simulink model "Autonomous_4x4_ML_Control"  (R2026a)
settings: Solver=FixedStepAuto  StopTime=10  FixedStep=0.01  MaxStep=.01  AbsTol=1e-6
PreLoadFcn:
  | % Load initialization data
  | 
  | sldemo_absdata;
undefined symbols (not defined in the file): DiscIntNeverNeededParam, g, m, m_vehicle, mu, RoadFrictionFactor, Rr, slip, v0
libraries: statsLibrary x1
CloseFcn:
  | % Close the plots that are still open
  | h = findobj(0, 'Name', 'ABS Speeds');
  | if ~isempty(h),
  |   close(h);
  | end;
  | 
  | h = findobj(0, 'Name', 'ABS Slip');
  | if ~isempty(h),
  |   close(h);
  | end;
  | 
  | % Clear initial conditions data to avoid cluttering the workspace
  | 
  | clear g v0 Rr Kf m PBmax TB I slip mu ctrl h;
Description:
  | Modeling an Anti-Lock Braking System (ABS)
  | 
  | *Summary*
  | 
  | This example describes a simple model for an Anti-Lock Braking System
  | (ABS). The model simulates the dynamic behavior of a vehicle
  | under hard braking conditions. The model represents a single wheel, which
  | may be replicated a number of times to create a model for a multi-wheel
  | vehicle.
  | 
  | This model uses the signal logging feature in Simulink(R). You log signals to the
  | MATLAB(R) workspace where you can analyze and view them. You can view
  | the code in sldemo_absbrakeplots.m to see how this is done.
  | 
  | In this model, the wheel speed is calculated in a separate component
  | named sldemo_wheelspeed_absbrake.
  | This component is then referenced using a Model block.  Note that both the
  | top model and the referenced model use a variable step solver, so Simulink
  | will track zero-crossings in the referenced model.
settings Model: FPTRunName=Active  ModifiedByFormat=The MathWorks, Inc.  ExtModeTrigMode=oneshot  ExtModeArmWhenConnect=off  ExtModeAutoUpdateStatusClock=off  Creator=The MathWorks, Inc.  LastModifiedBy=The MathWorks, Inc.
settings DataIOCC: TimeSaveName=time  SignalLoggingName=sldemo_absbrake_output
settings OptimizationCC: UseDivisionForNetSlopeComputation=on  InlineInvariantSignals=on  StateBitsets=on  DataBitsets=on  EfficientFloat2IntCast=on  BufferReusableBoundary=off
settings DebuggingCC: SignalInfNanChecking=warning  SaveWithParameterizedLinksMsg=none  SigSpecEnsureSampleTimeMsg=none  IntegerOverflowMsg=error  UniqueDataStoreMsg=error  BusObjectLabelMismatch=none  AssertControl=DisableAll  SubsystemReferenceDiagnosticForUnitTest=warning  SFUndirectedBroadcastEventsDiag=error  IntegerSaturationMsg=none
settings HardwareCC: ProdHWDeviceType=32-bit Generic  TargetBitPerPointer=64.0  TargetBitPerSizeT=64.0  TargetBitPerPtrDiffT=64.0  TargetLongLongMode=on  TargetIntDivRoundTo=Zero  TargetEndianess=LittleEndian  TargetWordSize=64.0  TargetHWDeviceType=MATLAB Host
settings SFSimCC: CompileTimeRecursionLimit=0.0  EnableRuntimeRecursion=off
settings RTWCC: SystemTargetFile=ert.tlc  Description=Embedded Coder
settings CodeAppCC: IgnoreTestpoints=on  MATLABFcnDesc=on
settings ERTTargetCC: EnableSignedLeftShifts=off  EnableSignedRightShifts=off  DynamicArrayContainerType=coder::array  UtilityFuncGeneration=Shared location  GenerateSampleERTMain=on  SupportAbsoluteTime=off  ParenthesesLevel=Standards  CastingMode=Standards  GenerateSharedConstants=off
settings SimscapeCC: SimscapeLogType=none  SimscapeNominalValues="[{\"value\":\"1\",\"unit\":\"A\"},{\"value\":\"1\",\"unit\":\"bar\"},{\"value\":\"1\",\"unit\":\"cm^2\"},{\"value\":\"1\",\"unit\":\"cm^3/s\"},{\"value\":\"1\",\"unit\":\"kJ/kg\"},{\"value\":\"1\",\"unit\":\"kW\"},{\"value\":\"1\",\"unit\":\"l\"},{\"value\":\"1\",\"unit\":\"N\"},{\"value\":\"1\",\"unit\":\"N*m\"},{\"value\":\"1\",\"unit\":\"V\"}]"  SimscapeLogDataHistory=5000.0

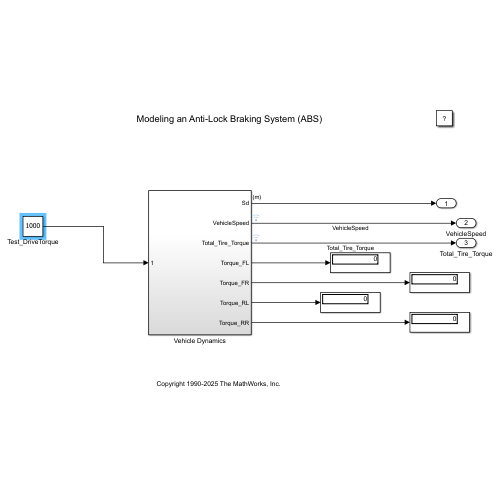
[thumbnail: Simulink's stored preview of the top-level diagram]
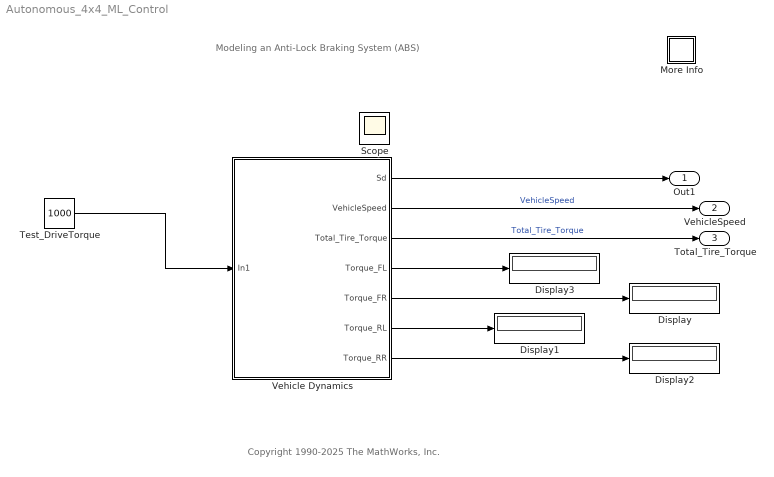
== system Autonomous_4x4_ML_Control ==
  note: Modeling an Anti-Lock Braking System (ABS)
  note: Copyright 1990-2025 The MathWorks, Inc.
  Display{,1..3} (4 alike) : Display
  More Info : Subsystem
      settings: OpenFcn=showExample('simulink_automotive/ModelingAnAntiLockBrakingSystemExample')
      mask Display: disp('?')
  Test_DriveTorque : Constant  Value=1000
  Vehicle Dynamics : Subsystem
  Out1 : Outport
  VehicleSpeed : Outport  Port=2
  Total_Tire_Torque : Outport  Port=3
  Scope : Scope
      settings: ActiveDisplayYMinimum=-8.8  ActiveDisplayYMaximum=79.2
  wires:
  Vehicle Dynamics/1(Sd) -> Out1/1
  Vehicle Dynamics/2(VehicleSpeed) -> VehicleSpeed/1  "VehicleSpeed"
  Vehicle Dynamics/3(Total_Tire_Torque) -> Total_Tire_Torque/1  "Total_Tire_Torque"
  Test_DriveTorque/1 -> Vehicle Dynamics/1(In1)
  Vehicle Dynamics/5(Torque_FR) -> Display/1
  Vehicle Dynamics/4(Torque_FL) -> Display3/1
  Vehicle Dynamics/6(Torque_RL) -> Display1/1
  Vehicle Dynamics/7(Torque_RR) -> Display2/1

== system Autonomous_4x4_ML_Control/More Info ==

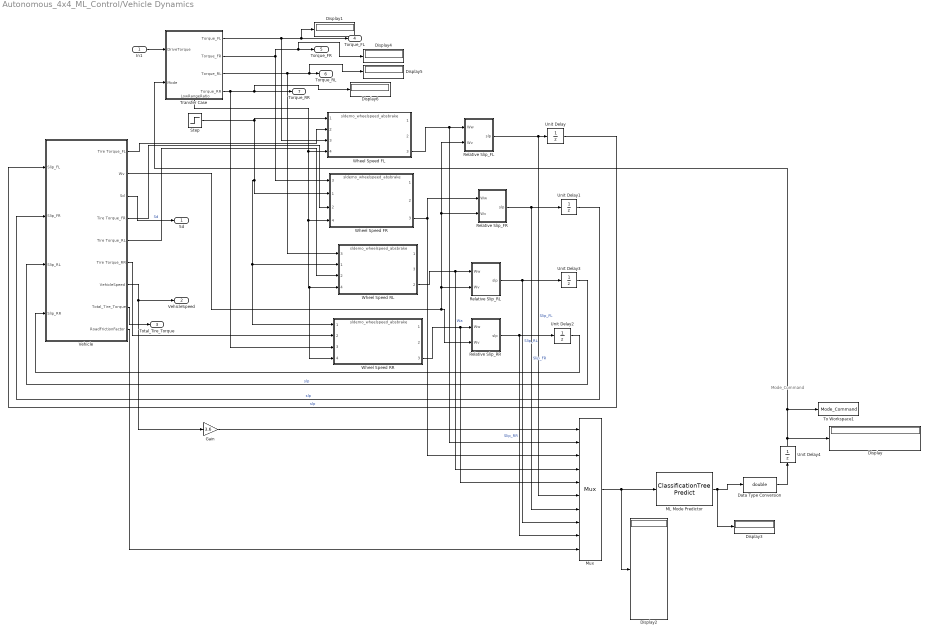
== system Autonomous_4x4_ML_Control/Vehicle Dynamics ==
  note: Mode_Command
  In1 : Inport
  Data Type Conversion : DataTypeConversion  OutDataTypeStr=double  SaturateOnIntegerOverflow=off  RndMeth=Floor
  Display{,1..6} (7 alike) : Display
  Gain : Gain  Gain=3.6
  ML Mode Predictor : statsLibrary/Classification/ClassificationTree Predict  TrainedLearner=MdlNum  ShowOutputScore=off  LabelDataTypeStr=Inherit: Inherit via back propagation  LabelOutMin=[]  LabelOutMax=[]  ScoreOutMin=[]  ScoreOutMax=[]  RawScoreOutMin=[]  RawScoreOutMax=[]  StoredEnumName=Mdl_enumLabels
  Mux : Mux  Inputs=10
  Relative Slip_FL : Subsystem
  Relative Slip_FR : Subsystem
  Relative Slip_RL : Subsystem
  Relative Slip_RR : Subsystem
  Step : Step  FinalValue=0  SampleTime=0
  To Workspace1 : ToWorkspace  VariableName=Mode_Command  SaveFormat=Timeseries  SampleTime=-1
  Transfer Case : Subsystem
      settings: PortSchema="{\"entries\":[{\"content\":{\"sides\":[{\"content\":{\"connectorIds\":[\"In1\",\"In2\"]},\"type\":\"ConnectorPlacement.EquallySpacedRectSide\",\"uuid\":\"0e4e5f2d-5f0e-4b2d-8d61-bd21c92eebc1\"},{\"content\":{\"connectorIds\":[\"Out1\",\"Out2\",\"Out3\",\"Out4\"],\"side\":\"RIGHT\"},\"type\":\"ConnectorPlacement.EquallySpacedRectSide\",\"uuid\":\"021f75cc-2385-4e1f-b164-196169dc630e\"},{\"content\":{\"side\":\"TOP\"},\"type\":\"ConnectorPlacement.EquallySpacedRectSide\",\"uuid\":\"94e51013-e54e-4a02-821d-d2a992c60f52\"},{\"content\":{\"connectorIds\":[\"Out5\"],\"side\":\"BOTTOM\"},\"type\":\"ConnectorPlacement.EquallySpacedRectSide\",\"uuid\":\"7324c2ae-c4f9-4421-b606-f82c567ae911\"}]},\"type\":\"ConnectorPlacement.EquallySpacedConnector\",\"uuid\":\"f212706d-3322-46ed-bdef-506210d0e9a5\"}],\"packageUris\":[\"http://schema.mathworks.com/mf0/Connector/R2020b\"],\"version\":\"1.0\"}"
  Unit Delay{,1..3} (4 alike) : UnitDelay  SampleTime=-1
  Unit Delay4 : UnitDelay  InitialCondition=1  SampleTime=-1
  "Vehicle  " : Subsystem
  Wheel Speed FL : ModelReference  ModelNameDialog=sldemo_wheelspeed_absbrake.slx  SimulationMode=Normal  ModelReferenceVersion=12.11
  Wheel Speed FR : ModelReference  ModelNameDialog=sldemo_wheelspeed_absbrake.slx  SimulationMode=Normal  ModelReferenceVersion=12.11
      settings: PortSchema="{\"entries\":[{\"content\":{\"sides\":[{\"content\":{\"connectorIds\":[\"In3\",\"In1\",\"In2\",\"In4\"]},\"type\":\"ConnectorPlacement.EquallySpacedRectSide\",\"uuid\":\"6283c4c6-a8cc-4cb2-bc3f-0488b786ccc3\"},{\"content\":{\"connectorIds\":[\"Out1\",\"Out2\",\"Out3\"],\"side\":\"RIGHT\"},\"type\":\"ConnectorPlacement.EquallySpacedRectSide\",\"uuid\":\"a506e2fe-25e7-45ab-91bb-1a7478d37f38\"},{\"content\":{\"side\":\"TOP\"},\"type\":\"ConnectorPlacement.EquallySpacedRectSide\",\"uuid\":\"8c371bb1-0729-467b-a425-cd217e166b59\"}]},\"type\":\"ConnectorPlacement.EquallySpacedConnector\",\"uuid\":\"2368ccbb-17fd-4c6b-9b61-3c68c899a72d\"}],\"packageUris\":[\"http://schema.mathworks.com/mf0/Connector/R2020b\"],\"version\":\"1.0\"}"
  Wheel Speed RL : ModelReference  ModelNameDialog=sldemo_wheelspeed_absbrake.slx  SimulationMode=Normal  ModelReferenceVersion=12.11
      settings: PortSchema="{\"entries\":[{\"content\":{\"sides\":[{\"content\":{\"connectorIds\":[\"In3\",\"In1\",\"In2\",\"In4\"]},\"type\":\"ConnectorPlacement.EquallySpacedRectSide\",\"uuid\":\"6283c4c6-a8cc-4cb2-bc3f-0488b786ccc3\"},{\"content\":{\"connectorIds\":[\"Out1\",\"Out3\",\"Out2\"],\"side\":\"RIGHT\"},\"type\":\"ConnectorPlacement.EquallySpacedRectSide\",\"uuid\":\"a506e2fe-25e7-45ab-91bb-1a7478d37f38\"},{\"content\":{\"side\":\"TOP\"},\"type\":\"ConnectorPlacement.EquallySpacedRectSide\",\"uuid\":\"8c371bb1-0729-467b-a425-cd217e166b59\"}]},\"type\":\"ConnectorPlacement.EquallySpacedConnector\",\"uuid\":\"2368ccbb-17fd-4c6b-9b61-3c68c899a72d\"}],\"packageUris\":[\"http://schema.mathworks.com/mf0/Connector/R2020b\"],\"version\":\"1.0\"}"
  Wheel Speed RR : ModelReference  ModelNameDialog=sldemo_wheelspeed_absbrake.slx  SimulationMode=Normal  ModelReferenceVersion=12.11
  Sd : Outport
  VehicleSpeed : Outport  Port=2
  Total_Tire_Torque : Outport  Port=3
  Torque_FL : Outport  Port=4
  Torque_FR : Outport  Port=5
  Torque_RL : Outport  Port=6
  Torque_RR : Outport  Port=7
  wires:
  "Vehicle  "/2(Wv) -> Relative Slip_RR/2(Wv), Relative Slip_RL/2(Wv), Relative Slip_FR/2(Wv), Relative Slip_FL/2(Wv)
  "Vehicle  "/1(Tire Torque_FL) -> Wheel Speed FL/2
  "Vehicle  "/3(Sd) -> Sd/1  "Sd"
  Relative Slip_FL/1(slp) -> Mux/6, Unit Delay/1  "Slip_FL"
  Unit Delay2/1 -> "Vehicle  "/4(Slip_RR)
  "Vehicle  "/4(Tire Torque_FR) -> Wheel Speed FR/2
  "Vehicle  "/5(Tire Torque_RL) -> Wheel Speed RL/2
  "Vehicle  "/6(Tire Torque_RR) -> Wheel Speed RR/2
  Relative Slip_FR/1(slp) -> Mux/7, Unit Delay1/1  "Slip_FR"
  Relative Slip_RL/1(slp) -> Mux/8, Unit Delay3/1  "Slip_RL"
  Relative Slip_RR/1(slp) -> Mux/9, Unit Delay2/1  "Slip_RR"
  Unit Delay/1 -> "Vehicle  "/1(Slip_FL)  "slp"
  Unit Delay1/1 -> "Vehicle  "/2(Slip_FR)  "slp"
  Unit Delay3/1 -> "Vehicle  "/3(Slip_RL)  "slp"
  Step/1 -> Wheel Speed RR/1, Wheel Speed RL/1, Wheel Speed FR/1, Wheel Speed FL/1
  "Vehicle  "/7(VehicleSpeed) -> VehicleSpeed/1, Gain/1
  "Vehicle  "/8(Total_Tire_Torque) -> Total_Tire_Torque/1
  In1/1 -> Transfer Case/1(DriveTorque)
  Transfer Case/1(Torque_FL) -> Display1/1, Torque_FL/1, Wheel Speed FL/3
  Transfer Case/2(Torque_FR) -> Display4/1, Torque_FR/1, Wheel Speed FR/3
  Transfer Case/3(Torque_RL) -> Wheel Speed RL/3, Display5/1, Torque_RL/1
  Transfer Case/4(Torque_RR) -> Wheel Speed RR/3, Display6/1, Torque_RR/1
  Transfer Case/5(LowRangeRatio) -> Wheel Speed RR/4, Wheel Speed RL/4, Wheel Speed FR/4, Wheel Speed FL/4
  Gain/1 -> Mux/1
  Wheel Speed FL/3 -> Mux/2, Relative Slip_FL/1(Ww)
  Wheel Speed FR/3 -> Mux/3, Relative Slip_FR/1(Ww)
  Wheel Speed RL/2 -> Mux/4, Relative Slip_RL/1(Ww)  "Wa"
  Wheel Speed RR/3 -> Mux/5, Relative Slip_RR/1(Ww)
  Mux/1 -> Display2/1, ML Mode Predictor/1
  "Vehicle  "/9(RoadFrictionFactor) -> Mux/10
  ML Mode Predictor/1 -> Display3/1, Data Type Conversion/1
  Data Type Conversion/1 -> Unit Delay4/1
  Unit Delay4/1 -> To Workspace1/1, Transfer Case/2(Mode), Display/1

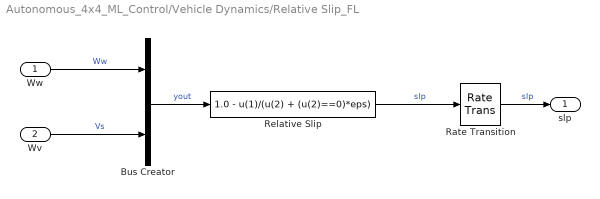
== system Autonomous_4x4_ML_Control/Vehicle Dynamics/Relative Slip_FL ==
  Ww : Inport
  Wv : Inport  Port=2
  Bus Creator : BusCreator  Inputs=2
  Rate Transition : RateTransition  OutPortSampleTimeOpt=Inherit
  Relative Slip : Fcn  Expr=1.0 - u(1)/(u(2) + (u(2)==0)*eps)
  slp : Outport
  wires:
  Bus Creator/1 -> Relative Slip/1  "yout"
  Relative Slip/1 -> Rate Transition/1  "slp"
  Ww/1 -> Bus Creator/1  "Ww"
  Wv/1 -> Bus Creator/2  "Vs"
  Rate Transition/1 -> slp/1  "slp"

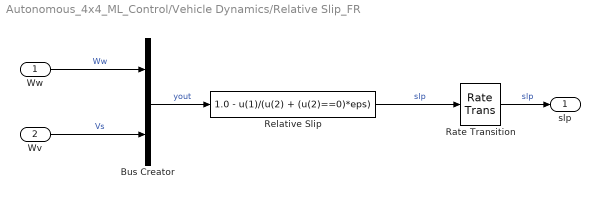
== system Autonomous_4x4_ML_Control/Vehicle Dynamics/Relative Slip_FR ==
  Ww : Inport
  Wv : Inport  Port=2
  Bus Creator : BusCreator  Inputs=2
  Rate Transition : RateTransition  OutPortSampleTimeOpt=Inherit
  Relative Slip : Fcn  Expr=1.0 - u(1)/(u(2) + (u(2)==0)*eps)
  slp : Outport
  wires:
  Bus Creator/1 -> Relative Slip/1  "yout"
  Relative Slip/1 -> Rate Transition/1  "slp"
  Ww/1 -> Bus Creator/1  "Ww"
  Wv/1 -> Bus Creator/2  "Vs"
  Rate Transition/1 -> slp/1  "slp"

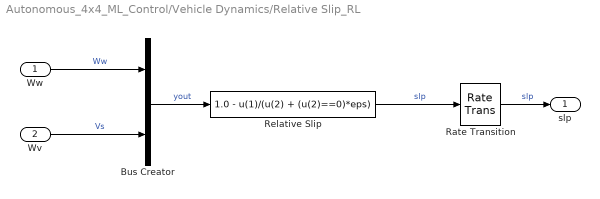
== system Autonomous_4x4_ML_Control/Vehicle Dynamics/Relative Slip_RL ==
  Ww : Inport
  Wv : Inport  Port=2
  Bus Creator : BusCreator  Inputs=2
  Rate Transition : RateTransition  OutPortSampleTimeOpt=Inherit
  Relative Slip : Fcn  Expr=1.0 - u(1)/(u(2) + (u(2)==0)*eps)
  slp : Outport
  wires:
  Bus Creator/1 -> Relative Slip/1  "yout"
  Relative Slip/1 -> Rate Transition/1  "slp"
  Ww/1 -> Bus Creator/1  "Ww"
  Wv/1 -> Bus Creator/2  "Vs"
  Rate Transition/1 -> slp/1  "slp"

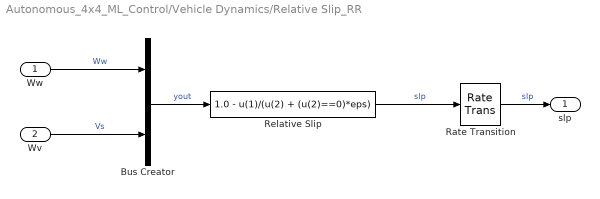
== system Autonomous_4x4_ML_Control/Vehicle Dynamics/Relative Slip_RR ==
  Ww : Inport
  Wv : Inport  Port=2
  Bus Creator : BusCreator  Inputs=2
  Rate Transition : RateTransition  OutPortSampleTimeOpt=Inherit
  Relative Slip : Fcn  Expr=1.0 - u(1)/(u(2) + (u(2)==0)*eps)
  slp : Outport
  wires:
  Bus Creator/1 -> Relative Slip/1  "yout"
  Relative Slip/1 -> Rate Transition/1  "slp"
  Ww/1 -> Bus Creator/1  "Ww"
  Wv/1 -> Bus Creator/2  "Vs"
  Rate Transition/1 -> slp/1  "slp"

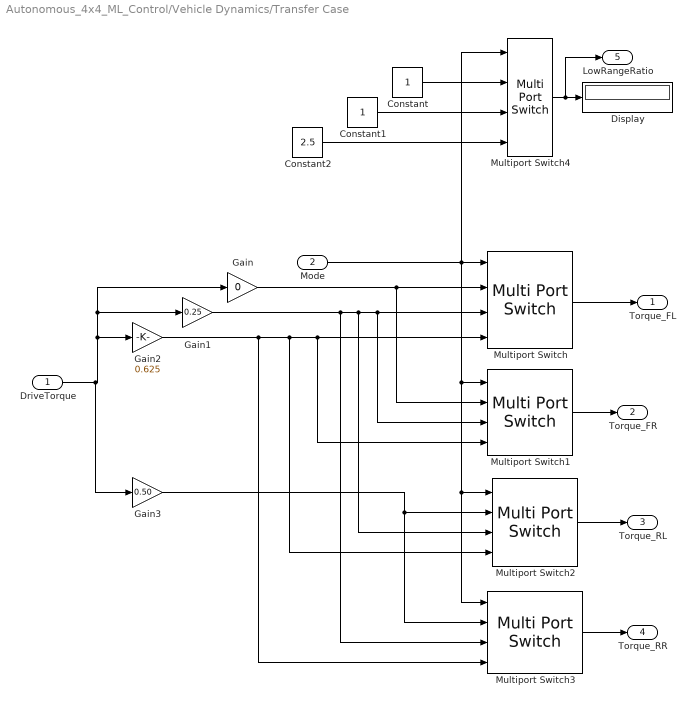
== system Autonomous_4x4_ML_Control/Vehicle Dynamics/Transfer Case ==
  DriveTorque : Inport
  Mode : Inport  Port=2  OutDataTypeStr=double  PortDimensions=1  LockScale=on
  Constant : Constant
  Constant1 : Constant
  Constant2 : Constant  Value=2.5
  Display : Display
  Gain : Gain  Gain=0
  Gain1 : Gain  Gain=0.25
  Gain2 : Gain  Gain=0.625
  Gain3 : Gain  Gain=0.50
  Multiport Switch{,1..4} (5 alike) : MultiPortSwitch  SaturateOnIntegerOverflow=off  InputSameDT=off
  Torque_FL : Outport
  Torque_FR : Outport  Port=2
  Torque_RL : Outport  Port=3
  Torque_RR : Outport  Port=4
  LowRangeRatio : Outport  Port=5
  wires:
  Multiport Switch/1 -> Torque_FL/1
  Multiport Switch1/1 -> Torque_FR/1
  Mode/1 -> Multiport Switch3/1, Multiport Switch2/1, Multiport Switch1/1, Multiport Switch/1, Multiport Switch4/1
  Multiport Switch2/1 -> Torque_RL/1
  Multiport Switch3/1 -> Torque_RR/1
  Gain/1 -> Multiport Switch1/2, Multiport Switch/2
  Gain1/1 -> Multiport Switch3/3, Multiport Switch2/3, Multiport Switch1/3, Multiport Switch/3
  Gain3/1 -> Multiport Switch3/2, Multiport Switch2/2
  Gain2/1 -> Multiport Switch3/4, Multiport Switch2/4, Multiport Switch1/4, Multiport Switch/4
  DriveTorque/1 -> Gain3/1, Gain2/1, Gain1/1, Gain/1
  Constant/1 -> Multiport Switch4/2
  Constant1/1 -> Multiport Switch4/3
  Constant2/1 -> Multiport Switch4/4
  Multiport Switch4/1 -> LowRangeRatio/1, Display/1

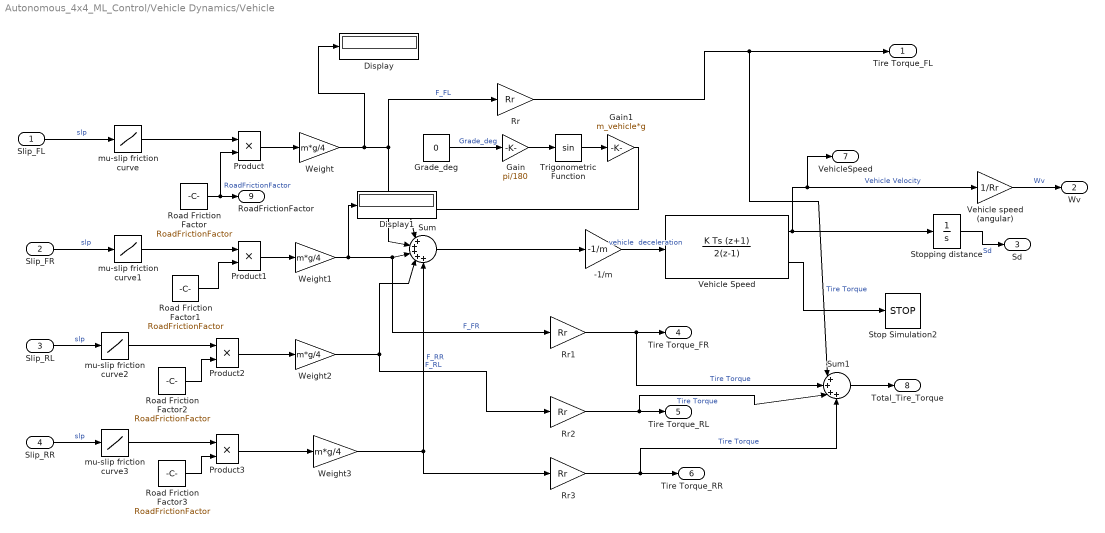
== system Autonomous_4x4_ML_Control/Vehicle Dynamics/Vehicle   ==
  Slip_FL : Inport
  Slip_FR : Inport  Port=2
  Slip_RL : Inport  Port=3
  Slip_RR : Inport  Port=4
  -1/m : Gain  Gain=-1/m  SaturateOnIntegerOverflow=on  OutDataTypeStr=Inherit: Same as input  ParamDataTypeStr=Inherit: Same as input
  Display : Display
  Display1 : Display
  Gain : Gain  Gain=pi/180
  Gain1 : Gain  Gain=m_vehicle*g
  Grade_deg : Constant  Value=0
  Product{,1..3} (4 alike) : Product
  Road Friction Factor{,1..3} (4 alike) : Constant  Value=RoadFrictionFactor
  Rr{,1..3} (4 alike) : Gain  Gain=Rr  SaturateOnIntegerOverflow=on  OutDataTypeStr=Inherit: Same as input  ParamDataTypeStr=Inherit: Same as input
  Stop Simulation2 : Stop
  Stopping distance : Integrator  UpperSaturationLimit=1000  LowerSaturationLimit=0
  Sum : Sum  Inputs=|+++++
  Sum1 : Sum  Inputs=|++++
  Trigonometric Function : Trigonometry
  Vehicle Speed : DiscreteIntegrator  IntegratorMethod=Integration: Trapezoidal  InitialCondition=v0  SampleTime=-1  LimitOutput=on  UpperSaturationLimit=1000  LowerSaturationLimit=0  ShowSaturationPort=on  ICPrevOutput=DiscIntNeverNeededParam  ICPrevScaledInput=DiscIntNeverNeededParam
  Vehicle speed (angular) : Gain  Gain=1/Rr  SaturateOnIntegerOverflow=on  OutDataTypeStr=Inherit: Same as input  ParamDataTypeStr=Inherit: Same as input
  Weight{,1..3} (4 alike) : Gain  Gain=m*g/4  SaturateOnIntegerOverflow=on  OutDataTypeStr=Inherit: Same as input  ParamDataTypeStr=Inherit: Same as input
  mu-slip friction curve{,1..3} (4 alike) : Lookup_n-D  NumberOfTableDimensions=1  BreakpointsForDimension1=slip  Table=mu  SaturateOnIntegerOverflow=on
  Tire Torque_FL : Outport  Unit=N*m
  Wv : Outport  Port=2  Unit=rad/sec
  Sd : Outport  Port=3  Unit=m
  Tire Torque_FR : Outport  Port=4  Unit=N*m
  Tire Torque_RL : Outport  Port=5  Unit=N*m
  Tire Torque_RR : Outport  Port=6  Unit=N*m
  VehicleSpeed : Outport  Port=7
  Total_Tire_Torque : Outport  Port=8
  RoadFrictionFactor : Outport  Port=9
  wires:
  Slip_FL/1 -> mu-slip friction curve/1  "slp"
  Rr/1 -> Sum1/1, Tire Torque_FL/1  "Tire Torque"
  -1/m/1 -> Vehicle Speed/1  "vehicle  deceleration"
  Vehicle speed (angular)/1 -> Wv/1  "Wv"
  Stopping distance/1 -> Sd/1  "Sd"
  Weight/1 -> Display/1, Rr/1, Sum/2  "F_FL"
  Vehicle Speed/1 -> VehicleSpeed/1, Vehicle speed (angular)/1, Stopping distance/1  "Vehicle Velocity"
  Vehicle Speed/2 -> Stop Simulation2/1
  Slip_FR/1 -> mu-slip friction curve1/1  "slp"
  Slip_RL/1 -> mu-slip friction curve2/1  "slp"
  Slip_RR/1 -> mu-slip friction curve3/1  "slp"
  mu-slip friction curve1/1 -> Product1/1
  mu-slip friction curve3/1 -> Product3/1
  mu-slip friction curve2/1 -> Product2/1
  Weight1/1 -> Display1/1, Sum/3, Rr1/1  "F_FR"
  Weight3/1 -> Sum/5, Rr3/1  "F_RR"
  Weight2/1 -> Sum/4, Rr2/1  "F_RL"
  Sum/1 -> -1/m/1
  Rr3/1 -> Sum1/4, Tire Torque_RR/1  "Tire Torque"
  Rr2/1 -> Sum1/3, Tire Torque_RL/1  "Tire Torque"
  Rr1/1 -> Sum1/2, Tire Torque_FR/1  "Tire Torque"
  Grade_deg/1 -> Gain/1  "Grade_deg"
  Gain/1 -> Trigonometric Function/1
  Trigonometric Function/1 -> Gain1/1
  Gain1/1 -> Sum/1
  mu-slip friction curve/1 -> Product/1
  Road Friction Factor/1 -> RoadFrictionFactor/1, Product/2  "RoadFrictionFactor"
  Product/1 -> Weight/1
  Product2/1 -> Weight2/1
  Product3/1 -> Weight3/1
  Product1/1 -> Weight1/1
  Road Friction Factor3/1 -> Product3/2
  Road Friction Factor2/1 -> Product2/2
  Road Friction Factor1/1 -> Product1/2
  Sum1/1 -> Total_Tire_Torque/1
